simulink model "Q5_MPPT"  (R2024b)
settings: Solver=FixedStepDiscrete  StartTime=0.0  StopTime=5  FixedStep=5e-6  RelTol=1e-3
PreLoadFcn:
  | % --- Q5 init variables (runs when model loads/initializes) ---
  | t = [0 2.5 5]';
  | G = [1000 400 1000]';
  | G_ts = timeseries(G,t);
  | assignin('base','G_ts',G_ts);
  | 
  | if ~evalin('base','exist(''mppt_mode'',''var'')')
  |     assignin('base','mppt_mode',1);
  | end
values from neighbouring files (symbols this model uses):
  mppt_mode = 2    [run_Q5.m]
libraries: spsSeriesRLCBranchLib x5, spsIdealSwitchLib x2, simulink x2, spsVoltageMeasurementLib x2, spsCurrentMeasurementLib x1, spsDiodeLib x1, spsIGBTDiodeLib x1, spsPVArrayLib x1, sps_lib x1
settings Model: Creator=mehme  LastModifiedBy=mehme
settings DataIOCC: ReturnWorkspaceOutputs=off

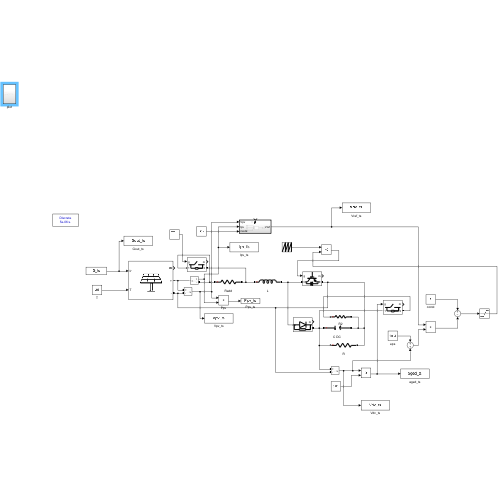
[thumbnail: Simulink's stored preview of the top-level diagram]
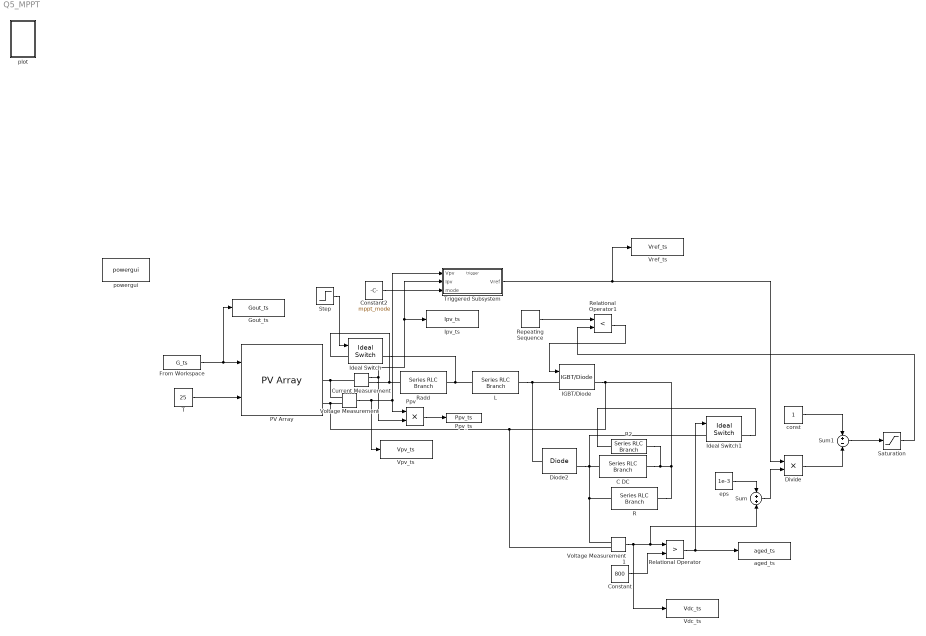
== system Q5_MPPT ==
  "C DC " : spsSeriesRLCBranchLib/Series RLC Branch  LConnTagsString=__new0  RConnTagsString=__new0  BranchType=C  Resistance=1  Inductance=2e-3  SetiL0=off  InitialCurrent=0  Capacitance=2e-3  Setx0=off  InitialVoltage=0  Measurements=None
  Constant : Constant  Value=800
  Constant2 : Constant  Value=mppt_mode
  Current Measurement : spsCurrentMeasurementLib/Current Measurement  PhasorSimulation=off  OutputType=Complex  PSBequivalent=0
  Diode2 : spsDiodeLib/Diode  Ron=0.001  Lon=0  Vf=0.8  IC=0  UseSnubber=0  Rs=500  Cs=250e-9  Measurements=on
  Divide : Product
  From Workspace : FromWorkspace  VariableName=G_ts  SampleTime=2e-4
  Gout_ts : ToWorkspace  VariableName=Gout_ts  SaveFormat=Timeseries  SampleTime=-1
  IGBT/Diode : spsIGBTDiodeLib/IGBT//Diode  Ron=1e-3  Rs=1e5  Cs=inf  Measurements=on
  Ideal Switch : spsIdealSwitchLib/Ideal Switch  Ron=0.001  Lon=0  IC=0  Rs=1e5  Cs=inf  Measurements=on
  Ideal Switch1 : spsIdealSwitchLib/Ideal Switch  Ron=0.001  Lon=0  IC=0  Rs=1e5  Cs=inf  Measurements=on
  Ipv_ts : ToWorkspace  VariableName=Ipv_ts  SaveFormat=Timeseries  SampleTime=-1
  L : spsSeriesRLCBranchLib/Series RLC Branch  LConnTagsString=__new0  RConnTagsString=__new0  BranchType=L  Resistance=1  Inductance=2e-3  SetiL0=off  InitialCurrent=0  Capacitance=1e-6  Setx0=off  InitialVoltage=0  Measurements=None
  PV Array : spsPVArrayLib/PV Array  Npar=11  Nser=22  PlotType=array @ 1000 W/m2 & specified temperatures  S_vec="[ 1000  500  100 ]"  Temp_C_vec="[ 45 25  ]"  ModuleName=User-defined  PlotWhenSelected=off  Pm=213.15  Ncell=60  Voc=36.3  Isc=7.84  Vm=29  Im=7.35  beta_Voc_pc=-0.36099  alpha_Isc_pc=0.102  beta_Voc=-0.13104  alpha_Isc=0.0079968  IL=7.8654  I0=2.9273e-10  nI=0.98119  Rsh=313.0553  Rs=0.39381  RobustModel=off  RobustCellTemperature=313.3991  BAL=on  Tc=1e-6  Tfilter=5e-5
  Ppv : Product
  Ppv_ts : ToWorkspace  VariableName=Ppv_ts  SaveFormat=Timeseries  SampleTime=-1
  R : spsSeriesRLCBranchLib/Series RLC Branch  LConnTagsString=__new0  RConnTagsString=__new0  BranchType=R  Resistance=10  Inductance=2e-3  SetiL0=off  InitialCurrent=0  Capacitance=2e-3  Setx0=off  InitialVoltage=0  Measurements=None
  R2 : spsSeriesRLCBranchLib/Series RLC Branch  LConnTagsString=__new0  RConnTagsString=__new0  BranchType=R  Resistance=20  Inductance=2e-3  SetiL0=off  InitialCurrent=0  Capacitance=1e-6  Setx0=off  InitialVoltage=0  Measurements=None
  Radd : spsSeriesRLCBranchLib/Series RLC Branch  LConnTagsString=__new0  RConnTagsString=__new0  BranchType=R  Resistance=0.08  Inductance=1e-3  SetiL0=off  InitialCurrent=0  Capacitance=1e-6  Setx0=off  InitialVoltage=0  Measurements=None
  Relational Operator : RelationalOperator  Operator=>  OutDataTypeStr=boolean  RndMeth=Simplest  InputSameDT=off
  Relational Operator1 : RelationalOperator  Operator=<  OutDataTypeStr=boolean  RndMeth=Simplest  InputSameDT=off
  Repeating Sequence : simulink/Sources/Repeating Sequence  rep_seq_t=[0 2e-4]  rep_seq_y=[0 1]
  Saturation : Saturate  UpperLimit=0.95  LowerLimit=0.05
  Step : Step  Time=2.5  Before=1  After=0  SampleTime=0
  Sum : Sum
  Sum1 : Sum  Inputs=+-
  T : Constant  Value=25
  Triggered Subsystem : Subsystem  TreatAsAtomicUnit=on
  Vdc_ts : ToWorkspace  VariableName=Vdc_ts  SaveFormat=Timeseries  SampleTime=-1
  Voltage Measurement : spsVoltageMeasurementLib/Voltage Measurement  PhasorSimulation=off  OutputType=Complex  PSBequivalent=0
  Voltage Measurement1 : spsVoltageMeasurementLib/Voltage Measurement  PhasorSimulation=off  OutputType=Complex  PSBequivalent=0
  Vpv_ts : ToWorkspace  VariableName=Vpv_ts  SaveFormat=Timeseries  SampleTime=-1
  Vref_ts : ToWorkspace  VariableName=Vref_ts  SaveFormat=Timeseries  SampleTime=-1
  aged_ts : ToWorkspace  VariableName=aged_ts  SaveFormat=Timeseries  SampleTime=-1
  const : Constant
  eps : Constant  Value=1e-3
  plot : Subsystem
  powergui : sps_lib/powergui  Priority=1  SimulationMode=Discrete  SampleTime=5e-6  frequency=60  Iterations=50  frequencyindice=0  Pbase=100e6  ErrMax=1e-4  UnitsV=kV  UnitsW=MW  buscounter=0  FunctionMessages=off  echomessages=off  EnableUseOfTLC=off  CurrentSourceSwitches=off  DisableSnubberDevices=off  DisableRonSwitches=off  DisableVfSwitches=off  DisplayEquations=off  AutomaticDiscreteSolvers=off  SolverType=Tustin/Backward Euler (TBE)  Interpol=off  ExternalGateDelay=off  methode=off  Ts=100  x0status=blocks  SPID=on  SwTol=0  HookPort=off  NonlinearTolerance=1e-4  nMaxIteration=100  ContinueOnMaxIteration=off  RestoreLinks=warning  ResistiveCurrentMeasurement=off  Frange=[0:2:500]  Ylog=off  Xlog=on  ShowGrid=off  save=off  variable=ZData  structure=0  ZoomFFT=off  StartTime=0.0  cycles=1  DisplayStyle=1  fundamental=60  FreqAxis=off  MaxFrequency=1000  frequencyindicesteady=1  RmsSteady=1  display=off
  wires:
  T/1 -> PV Array/2
  From Workspace/1 -> Gout_ts/1, PV Array/1
  Step/1 -> Ideal Switch/1
  Voltage Measurement/1 -> Ppv/1, Triggered Subsystem/1(Vpv), Vpv_ts/1
  Current Measurement/1 -> Ipv_ts/1, Triggered Subsystem/2(Ipv), Ppv/2
  Constant/1 -> Relational Operator/2
  Relational Operator/1 -> aged_ts/1, Ideal Switch1/1
  Repeating Sequence/1 -> Relational Operator1/1
  Relational Operator1/1 -> IGBT/Diode/1
  Constant2/1 -> Triggered Subsystem/3(mode)
  Triggered Subsystem/1(Vref) -> Vref_ts/1, Divide/1
  Sum/1 -> Divide/2
  eps/1 -> Sum/1
  const/1 -> Sum1/1
  Divide/1 -> Sum1/2
  Sum1/1 -> Saturation/1
  Saturation/1 -> Relational Operator1/2
  Voltage Measurement1/1 -> Vdc_ts/1, Sum/2, Relational Operator/1
  Ppv/1 -> Ppv_ts/1
  connections:
  Current Measurement/LConn1 -- Voltage Measurement/LConn1 -- PV Array/RConn1
  Voltage Measurement/LConn2 -- R2/RConn1 -- "C DC "/RConn1 -- R/RConn1 -- IGBT/Diode/RConn1 -- Voltage Measurement1/LConn2 -- PV Array/RConn2
  Current Measurement/RConn1 -- Ideal Switch/LConn1 -- Radd/LConn1
  Radd/RConn1 -- Ideal Switch/RConn1 -- L/LConn1
  L/RConn1 -- Diode2/LConn1 -- IGBT/Diode/LConn1
  Diode2/RConn1 -- Ideal Switch1/LConn1 -- Voltage Measurement1/LConn1 -- R/LConn1 -- "C DC "/LConn1
  Ideal Switch1/RConn1 -- R2/LConn1

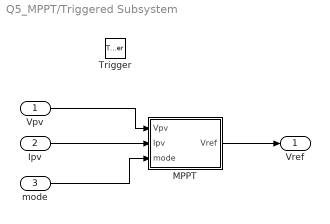
== system Q5_MPPT/Triggered Subsystem ==
  Vpv : Inport
  Ipv : Inport  Port=2
  mode : Inport  Port=3
  Trigger : TriggerPort  VariantControl=(inherit)
  MPPT : MATLAB Function  TreatAsAtomicUnit=on
  Vref : Outport
  wires:
  Vpv/1 -> MPPT/1(Vpv)
  Ipv/1 -> MPPT/2(Ipv)
  mode/1 -> MPPT/3(mode)
  MPPT/1(Vref) -> Vref/1

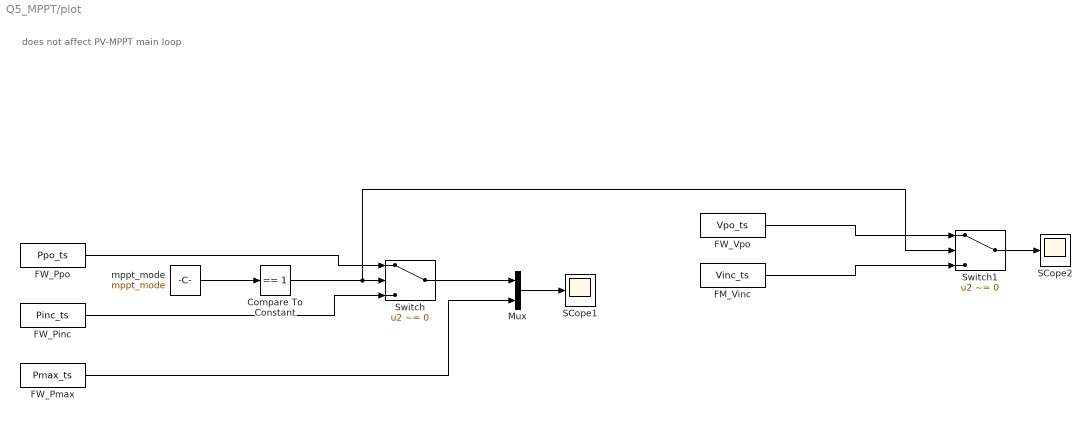
== system Q5_MPPT/plot ==
  note: does not affect PV-MPPT main loop
  Compare To Constant : simulink/Logic and Bit Operations/Compare To Constant  relop===  const=1  OutDataTypeStr=boolean
  FM_Vinc : FromWorkspace  VariableName=Vinc_ts  SampleTime=1e-3
  FW_Pinc : FromWorkspace  VariableName=Pinc_ts  SampleTime=1e-3
  FW_Pmax : FromWorkspace  VariableName=Pmax_ts  SampleTime=1e-3
  FW_Ppo : FromWorkspace  VariableName=Ppo_ts  SampleTime=1e-3
  FW_Vpo : FromWorkspace  VariableName=Vpo_ts  SampleTime=1e-3
  Mux : Mux  Inputs=2
  SCope1 : Scope
  SCope2 : Scope
  Switch : Switch  Criteria=u2 ~= 0  SaturateOnIntegerOverflow=off  InputSameDT=off
  Switch1 : Switch  Criteria=u2 ~= 0  SaturateOnIntegerOverflow=off  InputSameDT=off
  mppt_mode : Constant  Value=mppt_mode
  wires:
  FW_Pmax/1 -> Mux/2
  Compare To Constant/1 -> Switch1/2, Switch/2
  FW_Vpo/1 -> Switch1/1
  FW_Pinc/1 -> Switch/3
  Switch1/1 -> SCope2/1
  FM_Vinc/1 -> Switch1/3
  Switch/1 -> Mux/1
  mppt_mode/1 -> Compare To Constant/1
  Mux/1 -> SCope1/1
  FW_Ppo/1 -> Switch/1

== matlab function Q5_MPPT/Triggered Subsystem/MPPT ==
  data: Vpv input; Vref output; Ipv input; mode input
function Vref = MPPT(Vpv, Ipv, mode)
% mode: 1 = Adaptive P&O, 2 = Incremental Conductance

Vmin = 500; 
Vmax = 800;

% Adaptive P&O params
Ks    = 0.01;
dVmin = 0.2;
dVmax = 10;

% InC params
dVfix   = 1.0;
epsCond = 0.002;
Pdb     = 50;
Vdb     = 0.2;
kdrift  = 0.02;

persistent Vref_k Vprev Iprev Pprev
if isempty(Vref_k)
    Vref_k = 650;
    Vprev  = Vpv;
    Iprev  = Ipv;
    Pprev  = Vpv*Ipv;
end

P   = Vpv*Ipv;
dV  = Vpv - Vprev;
dI  = Ipv - Iprev;
dP  = P   - Pprev;

eps = 1e-6;

if mode == 1
    slope = dP/(dV + eps);
    dVstep = Ks*abs(slope);
    if dVstep < dVmin, dVstep = dVmin; end
    if dVstep > dVmax, dVstep = dVmax; end

    if dP > 0
        if dV >= 0
            Vref_k = Vref_k + dVstep;
        else
            Vref_k = Vref_k - dVstep;
        end
    else
        if dV >= 0
            Vref_k = Vref_k - dVstep;
        else
            Vref_k = Vref_k + dVstep;
        end
    end

else
    if abs(dV) < eps
        if abs(dI) > eps
            Vref_k = Vref_k + sign(dI)*dVfix;
        end
    else
        incCond = dI/(dV + eps);
        err = incCond + Ipv/(Vpv + eps);

        if err > epsCond
            Vref_k = Vref_k + dVfix;
        elseif err < -epsCond
            Vref_k = Vref_k - dVfix;
        else
            if abs(dP) < Pdb && abs(dV) < Vdb
                Vref_k = Vref_k + kdrift*(Vpv - Vref_k);
            end
        end
    end
end

if Vref_k < Vmin, Vref_k = Vmin; end
if Vref_k > Vmax, Vref_k = Vmax; end

Vref = Vref_k;

Vprev = Vpv;
Iprev = Ipv;
Pprev = P;
end
